simulink model "CurrentHysteresis_Control"  (R2023b)
settings: Solver=ode23  StartTime=0.0  StopTime=2  MaxStep=1e-5  RelTol=1e-3
model workspace: external: MATLAB File D:\Simulink\Study\PMSM建模第三章\CurrentHysteresis_Control_Params.m (data not in the file)
values from neighbouring files (symbols this model uses):
  B = 0.008    [CurrentHysteresis_Control_Params.m]    (also in Foc_Params.m; VF_Params.m)
  J = 0.0008    [CurrentHysteresis_Control_Params.m]    (also in Foc_Params.m = 0.003; VF_Params.m = 0.003)
  Pn = 4    [CurrentHysteresis_Control_Params.m]    (also in Foc_Params.m; VF_Params.m)
  R = 2.875    [CurrentHysteresis_Control_Params.m]    (also in Foc_Params.m = 0.958; VF_Params.m = 0.958)
libraries: spsControlledVoltageSourceLib x4, spsPermanentMagnetSynchronousMachineLib x2, slpidlib x1, sps_lib x1
settings Model: Creator=123  LastModifiedBy=123

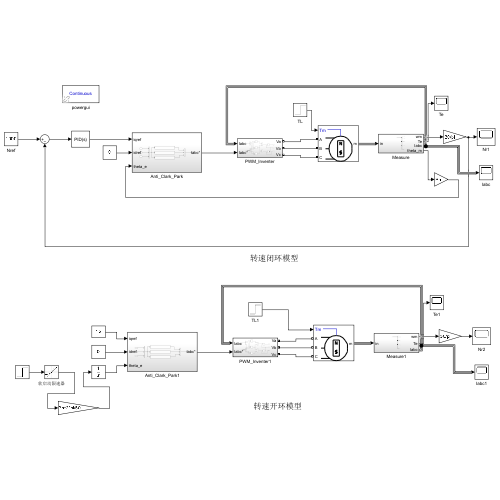
[thumbnail: Simulink's stored preview of the top-level diagram]
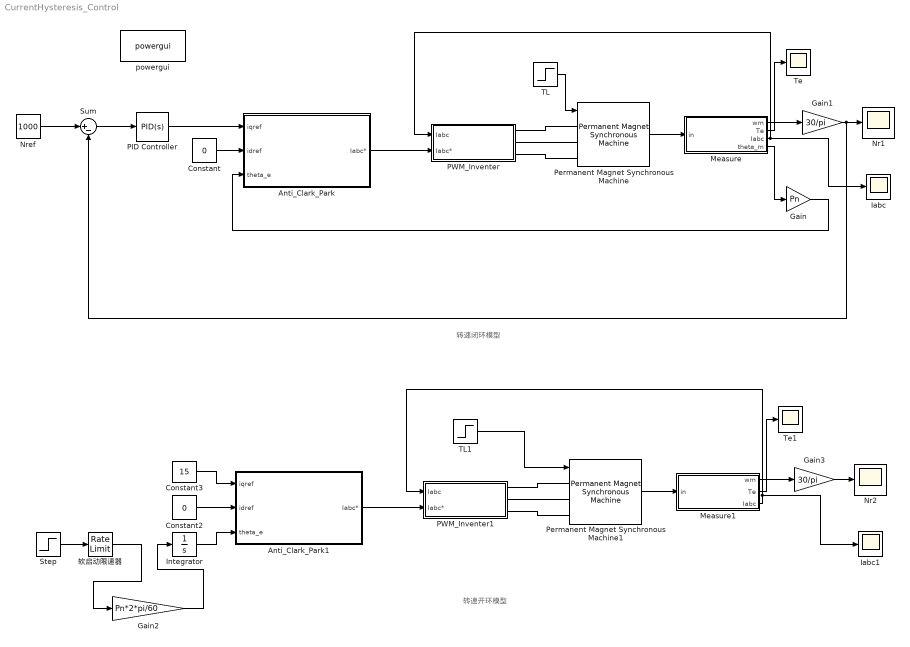
== system CurrentHysteresis_Control ==
  note: 转速开环模型
  note: 转速闭环模型
  Anti_Clark_Park : Subsystem
  Anti_Clark_Park1 : Subsystem
  Constant : Constant  Value=0
  Constant2 : Constant  Value=0
  Constant3 : Constant  Value=15
  Gain : Gain  Gain=Pn
  Gain1 : Gain  Gain=30/pi
  Gain2 : Gain  Gain=Pn*2*pi/60
  Gain3 : Gain  Gain=30/pi
  Iabc : Scope
  Iabc1 : Scope
  Integrator : Integrator
  Measure : Subsystem
  Measure1 : Subsystem
  Nr1 : Scope
  Nr2 : Scope
  Nref : Constant  Value=1000
  PID Controller : slpidlib/PID Controller  Controller=PID  Form=Parallel  TimeDomain=Continuous-time  UseExternalTs=off  SampleTime=-1  IntegratorMethod=Forward Euler  FilterMethod=Forward Euler  ControllerParametersSource=internal  P=0.06  I=10  UseKiTs=off  D=0  N=100  UseFilter=on  TunerSelectOption=Transfer Function Based (PID Tuner App)  InitialConditionSource=internal  InitialConditionForIntegrator=0  InitialConditionForFilter=0  DifferentiatorICPrevScaledInput=0  ExternalReset=none  TrackingMode=off  Kt=1  LimitOutput=off  SatLimitsSource=internal  UpperSaturationLimit=inf  LowerSaturationLimit=-inf  LinearizeAsGain=on  AntiWindupMode=none  Kb=1  LimitIntegrator=off  UpperIntegratorSaturationLimit=inf  LowerIntegratorSaturationLimit=-inf  POutMin=[]  POutMax=[]  IOutMin=[]  IOutMax=[]  DOutMin=[]  DOutMax=[]  NOutMin=[]  NOutMax=[]  SumOutMin=[]  SumOutMax=[]  SaturationOutMin=[]  SaturationOutMax=[]  PParamMin=[]  PParamMax=[]  IParamMin=[]  IParamMax=[]  DParamMin=[]  DParamMax=[]  NParamMin=[]  NParamMax=[]  KbParamMin=[]  KbParamMax=[]  KtParamMin=[]  KtParamMax=[]  KbOutMin=[]  KbOutMax=[]  KtOutMin=[]  KtOutMax=[]  IntegratorOutMin=[]  IntegratorOutMax=[]  FilterOutMin=[]  FilterOutMax=[]  SumI1OutMin=[]  SumI1OutMax=[]  SumI2OutMin=[]  SumI2OutMax=[]  SumI3OutMin=[]  SumI3OutMax=[]  SumI4OutMin=[]  SumI4OutMax=[]  SumDOutMin=[]  SumDOutMax=[]  DifferentiatorOutMin=[]  DifferentiatorOutMax=[]  FilterDiffOutCoefMin=[]  FilterDiffOutCoefMax=[]  ReciprocalOutMin=[]  ReciprocalOutMax=[]  SumDenOutMin=[]  SumDenOutMax=[]  SumNumOutMin=[]  SumNumOutMax=[]  DivideOutMin=[]  DivideOutMax=[]  UdiffTsProdOutMin=[]  UdiffTsProdOutMax=[]  NTsProdOutMin=[]  NTsProdOutMax=[]  UintegralTsProdOutMin=[]  UintegralTsProdOutMax=[]  UngainTsProdOutMin=[]  UngainTsProdOutMax=[]  ClampingZeroOutDataTypeStr=Inherit: Inherit via back propagation  ClampingZeroOutMin=[]  ClampingZeroOutMax=[]  FilterDenConstantOutDataTypeStr=Inherit: Inherit via back propagation  FilterDenConstantOutMin=[]  FilterDenConstantOutMax=[]  PCopyOutDataTypeStr=Inherit: Inherit via back propagation  PCopyOutMin=[]  PCopyOutMax=[]  NCopyOutDataTypeStr=Inherit: Inherit via back propagation  NCopyOutMin=[]  NCopyOutMax=[]  IntegratorContinuousStateAttributes=''  IntegratorStateMustResolveToSignalObject=off  IntegratorRTWStateStorageClass=Auto  FilterContinuousStateAttributes=''  FilterStateMustResolveToSignalObject=off  FilterRTWStateStorageClass=Auto  ParallelPVariant=InternalParameters  IdealPVariant=Disabled  IVariant=InternalParameters  DVariant=InternalParameters  IntegratorVariant=Continuous  SatVariant=Disabled  AWVariant=Passthrough  PCopyVariant=Disabled  TRVariant=Disabled  FdbkBlocksVariant=Forward  IdealPFdbkVariant=Disabled  SatFdbkVariant=Disabled  DerivativeFilterVariant=ContFilter  NVariant=InternalParameters  NCopyVariant=Disabled  FilterICVariant=InternalICsFilter  IntegratorICVariant=InternalICs  ExternalResetVariant=Disabled  TRSumVariant=Passthrough  SumFdbkVariant=Disabled  SumVariant=Sum_PID  TsampFilterVariant=InternalTs  TsampNgainVariant=Passthrough  TsampIntegralVariant=Disabled_SignalSpec  ExternalSaturationOutDataTypeStr=Inherit: Same as second input
  PWM_Inventer : Subsystem
  PWM_Inventer1 : Subsystem
  Permanent Magnet Synchronous Machine : spsPermanentMagnetSynchronousMachineLib/Permanent Magnet Synchronous Machine  NbPhases=3  FluxDistribution=Sinusoidal  RotorType=Round  MechanicalLoad=Torque Tm  PresetModel=No  ShowDetailedParameters=on  MeasurementBus=off  Resistance=R  Inductance=8.5e-3  dqInductances=[8.5e-3,8.5e-3]  La=Ld  MachineConstant=Flux linkage established by magnets (V.s)  Flux=flux  VoltageCst=126.966  TorqueCst=1.05  Flat=120  Mechanical=[J B Pn 0]  PolePairs=4  InitialConditions=[0,0, 0,0]  InitialConditions5ph=[0 0 0 0 0 0]  RefAngle=Aligned with phase A axis (original Park)  IterativeDiscreteModel=Trapezoidal non iterative  TsBlock=-1  TsPowergui=0
  Permanent Magnet Synchronous Machine1 : spsPermanentMagnetSynchronousMachineLib/Permanent Magnet Synchronous Machine  NbPhases=3  FluxDistribution=Sinusoidal  RotorType=Round  MechanicalLoad=Torque Tm  PresetModel=No  ShowDetailedParameters=on  MeasurementBus=off  Resistance=R  Inductance=8.5e-3  dqInductances=[8.5e-3,8.5e-3]  La=Ld  MachineConstant=Flux linkage established by magnets (V.s)  Flux=flux  VoltageCst=126.966  TorqueCst=1.05  Flat=120  Mechanical=[J B Pn 0]  PolePairs=4  InitialConditions=[0,0, 0,0]  InitialConditions5ph=[0 0 0 0 0 0]  RefAngle=Aligned with phase A axis (original Park)  IterativeDiscreteModel=Trapezoidal non iterative  TsBlock=-1  TsPowergui=0
  Step : Step  Time=0.1  After=1000  SampleTime=0
  Sum : Sum  Inputs=|+-
  TL : Step  Time=0.05  After=10  SampleTime=0
  TL1 : Step  After=10  SampleTime=0
  Te : Scope
  Te1 : Scope
  powergui : sps_lib/powergui  Priority=1  SimulationMode=Continuous  SampleTime=50e-6  frequency=60  Iterations=50  frequencyindice=0  Pbase=100e6  ErrMax=1e-4  UnitsV=kV  UnitsW=MW  buscounter=0  FunctionMessages=off  echomessages=off  EnableUseOfTLC=off  CurrentSourceSwitches=off  DisableSnubberDevices=off  DisableRonSwitches=off  DisableVfSwitches=off  DisplayEquations=off  AutomaticDiscreteSolvers=off  SolverType=Tustin/Backward Euler (TBE)  Interpol=off  ExternalGateDelay=off  methode=off  Ts=100  x0status=blocks  SPID=on  SwTol=0  HookPort=off  NonlinearTolerance=1e-4  nMaxIteration=100  ContinueOnMaxIteration=off  RestoreLinks=warning  ResistiveCurrentMeasurement=off  Frange=[0:2:500]  Ylog=off  Xlog=on  ShowGrid=off  save=off  variable=ZData  structure=0  ZoomFFT=off  StartTime=0.0  cycles=1  DisplayStyle=1  fundamental=60  FreqAxis=off  MaxFrequency=1000  frequencyindicesteady=1  RmsSteady=1  display=off
  软启动限速器 : RateLimiter  RisingSlewLimit=4000  FallingSlewLimit=-4000  SampleTimeMode=inherited
  wires:
  Nref/1 -> Sum/1
  Constant/1 -> Anti_Clark_Park/2(idref)
  Sum/1 -> PID Controller/1
  PID Controller/1 -> Anti_Clark_Park/1(iqref)
  Anti_Clark_Park/1(Iabc*) -> PWM_Inventer/2(Iabc*)
  Permanent Magnet Synchronous Machine/1 -> Measure/1(in)
  Gain1/1 -> Sum/2, Nr1/1
  Measure/1(wm) -> Gain1/1
  Measure/2(Te) -> Te/1
  Measure/4(theta_m) -> Gain/1
  Gain/1 -> Anti_Clark_Park/3(theta_e)
  Measure/3(Iabc) -> PWM_Inventer/1(Iabc), Iabc/1
  TL/1 -> Permanent Magnet Synchronous Machine/1
  Measure1/1(wm) -> Gain3/1
  Measure1/2(Te) -> Te1/1
  Gain3/1 -> Nr2/1
  Permanent Magnet Synchronous Machine1/1 -> Measure1/1(in)
  Measure1/3(Iabc) -> PWM_Inventer1/1(Iabc), Iabc1/1
  Anti_Clark_Park1/1(Iabc*) -> PWM_Inventer1/2(Iabc*)
  Step/1 -> 软启动限速器/1
  Integrator/1 -> Anti_Clark_Park1/3(theta_e)
  Constant2/1 -> Anti_Clark_Park1/2(idref)
  Constant3/1 -> Anti_Clark_Park1/1(iqref)
  软启动限速器/1 -> Gain2/1
  Gain2/1 -> Integrator/1
  TL1/1 -> Permanent Magnet Synchronous Machine1/1
  connections:
  PWM_Inventer/RConn1 -- Permanent Magnet Synchronous Machine/LConn1
  PWM_Inventer/RConn2 -- Permanent Magnet Synchronous Machine/LConn2
  PWM_Inventer/RConn3 -- Permanent Magnet Synchronous Machine/LConn3
  PWM_Inventer1/RConn3 -- Permanent Magnet Synchronous Machine1/LConn3
  PWM_Inventer1/RConn2 -- Permanent Magnet Synchronous Machine1/LConn2
  PWM_Inventer1/RConn1 -- Permanent Magnet Synchronous Machine1/LConn1

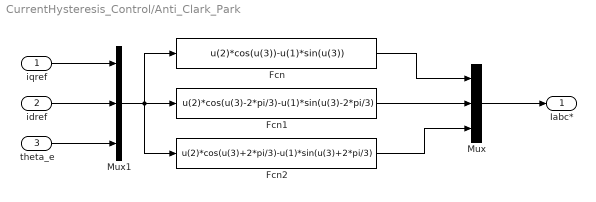
== system CurrentHysteresis_Control/Anti_Clark_Park ==
  iqref : Inport
  idref : Inport  Port=2
  theta_e : Inport  Port=3
  Fcn : Fcn  Expr=u(2)*cos(u(3))-u(1)*sin(u(3))
  Fcn1 : Fcn  Expr=u(2)*cos(u(3)-2*pi/3)-u(1)*sin(u(3)-2*pi/3)
  Fcn2 : Fcn  Expr=u(2)*cos(u(3)+2*pi/3)-u(1)*sin(u(3)+2*pi/3)
  Mux : Mux  Inputs=3
  Mux1 : Mux  Inputs=3
  Iabc* : Outport
  wires:
  Mux/1 -> Iabc*/1
  Fcn/1 -> Mux/1
  Fcn1/1 -> Mux/2
  Fcn2/1 -> Mux/3
  iqref/1 -> Mux1/1
  idref/1 -> Mux1/2
  theta_e/1 -> Mux1/3
  Mux1/1 -> Fcn1/1, Fcn/1, Fcn2/1

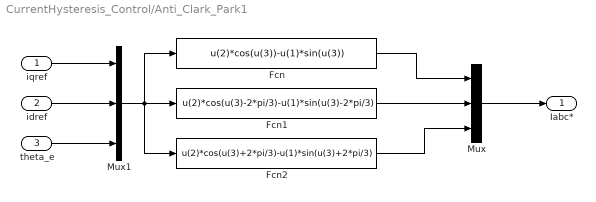
== system CurrentHysteresis_Control/Anti_Clark_Park1 ==
  iqref : Inport
  idref : Inport  Port=2
  theta_e : Inport  Port=3
  Fcn : Fcn  Expr=u(2)*cos(u(3))-u(1)*sin(u(3))
  Fcn1 : Fcn  Expr=u(2)*cos(u(3)-2*pi/3)-u(1)*sin(u(3)-2*pi/3)
  Fcn2 : Fcn  Expr=u(2)*cos(u(3)+2*pi/3)-u(1)*sin(u(3)+2*pi/3)
  Mux : Mux  Inputs=3
  Mux1 : Mux  Inputs=3
  Iabc* : Outport
  wires:
  Mux/1 -> Iabc*/1
  Fcn/1 -> Mux/1
  Fcn1/1 -> Mux/2
  Fcn2/1 -> Mux/3
  iqref/1 -> Mux1/1
  idref/1 -> Mux1/2
  theta_e/1 -> Mux1/3
  Mux1/1 -> Fcn1/1, Fcn/1, Fcn2/1

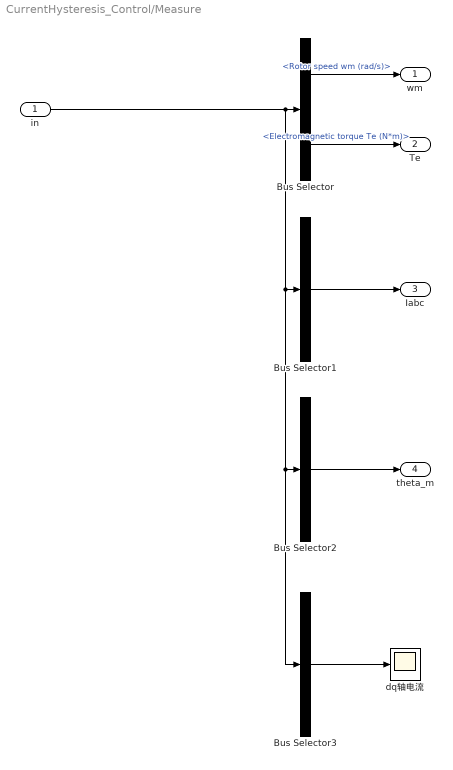
== system CurrentHysteresis_Control/Measure ==
  in : Inport
  Bus Selector : BusSelector  OutputSignals=Rotor speed wm (rad/s),Electromagnetic torque Te (N*m)
  Bus Selector1 : BusSelector  OutputSignals=Stator current is_a (A),Stator current is_b (A),Stator current is_c (A)  OutputAsBus=on
  Bus Selector2 : BusSelector  OutputSignals=Rotor angle thetam (rad)  OutputAsBus=on
  Bus Selector3 : BusSelector  OutputSignals=Stator current is_d (A),Stator current is_q (A)  OutputAsBus=on
  dq轴电流 : Scope
  wm : Outport
  Te : Outport  Port=2
  Iabc : Outport  Port=3
  theta_m : Outport  Port=4
  wires:
  in/1 -> Bus Selector3/1, Bus Selector2/1, Bus Selector1/1, Bus Selector/1
  Bus Selector/1 -> wm/1  "<Rotor speed wm (rad/s)>"
  Bus Selector/2 -> Te/1  "<Electromagnetic torque Te (N*m)>"
  Bus Selector1/1 -> Iabc/1
  Bus Selector2/1 -> theta_m/1
  Bus Selector3/1 -> dq轴电流/1

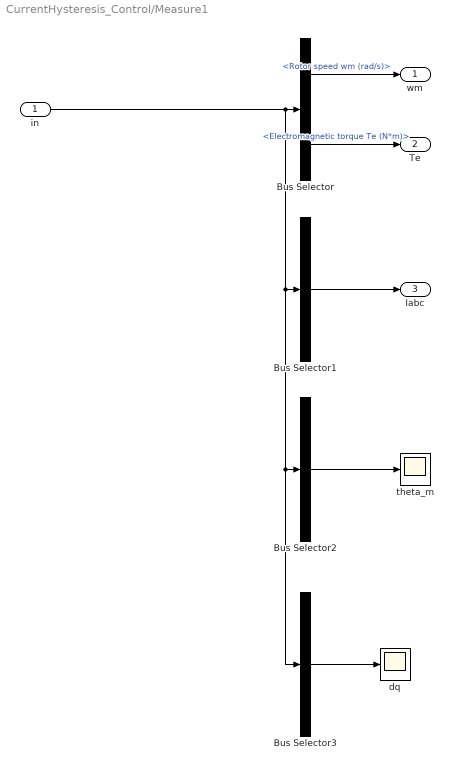
== system CurrentHysteresis_Control/Measure1 ==
  in : Inport
  Bus Selector : BusSelector  OutputSignals=Rotor speed wm (rad/s),Electromagnetic torque Te (N*m)
  Bus Selector1 : BusSelector  OutputSignals=Stator current is_a (A),Stator current is_b (A),Stator current is_c (A)  OutputAsBus=on
  Bus Selector2 : BusSelector  OutputSignals=Rotor angle thetam (rad)  OutputAsBus=on
  Bus Selector3 : BusSelector  OutputSignals=Stator current is_d (A),Stator current is_q (A)  OutputAsBus=on
  dq : Scope
  theta_m : Scope
  wm : Outport
  Te : Outport  Port=2
  Iabc : Outport  Port=3
  wires:
  in/1 -> Bus Selector3/1, Bus Selector2/1, Bus Selector1/1, Bus Selector/1
  Bus Selector/1 -> wm/1  "<Rotor speed wm (rad/s)>"
  Bus Selector/2 -> Te/1  "<Electromagnetic torque Te (N*m)>"
  Bus Selector1/1 -> Iabc/1
  Bus Selector2/1 -> theta_m/1
  Bus Selector3/1 -> dq/1

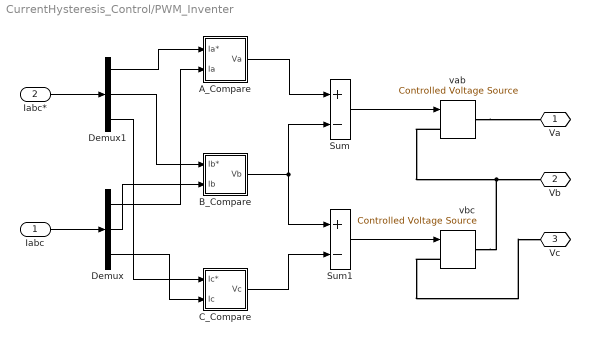
== system CurrentHysteresis_Control/PWM_Inventer ==
  Iabc : Inport
  Iabc* : Inport  Port=2
  A_Compare : Subsystem
  B_Compare : Subsystem
  C_Compare : Subsystem
  Demux : Demux  Outputs=3
  Demux1 : Demux  Outputs=3
  Sum : Sum  Inputs=+-
  Sum1 : Sum  Inputs=+-
  vab : spsControlledVoltageSourceLib/Controlled Voltage Source  Initialize=on  Source_Type=AC  Amplitude=0  Phase=0  Frequency=0  Measurements=None
  vbc : spsControlledVoltageSourceLib/Controlled Voltage Source  Initialize=on  Source_Type=AC  Amplitude=0  Phase=0  Frequency=0  Measurements=None
  Va : PMIOPort  Side=Right
  Vb : PMIOPort  Port=2  Side=Right
  Vc : PMIOPort  Port=3  Side=Right
  wires:
  Iabc/1 -> Demux/1
  Iabc*/1 -> Demux1/1
  Demux1/1 -> A_Compare/1(Ia*)
  Demux1/2 -> B_Compare/1(Ib*)
  Demux1/3 -> C_Compare/1(Ic*)
  Demux/3 -> C_Compare/2(Ic)
  Demux/2 -> B_Compare/2(Ib)
  Demux/1 -> A_Compare/2(Ia)
  A_Compare/1(Va) -> Sum/1
  B_Compare/1(Vb) -> Sum1/1, Sum/2
  C_Compare/1(Vc) -> Sum1/2
  Sum/1 -> vab/1
  Sum1/1 -> vbc/1
  connections:
  vab/RConn1 -- Va/RConn1
  vab/LConn1 -- vbc/RConn1 -- Vb/RConn1
  vbc/LConn1 -- Vc/RConn1

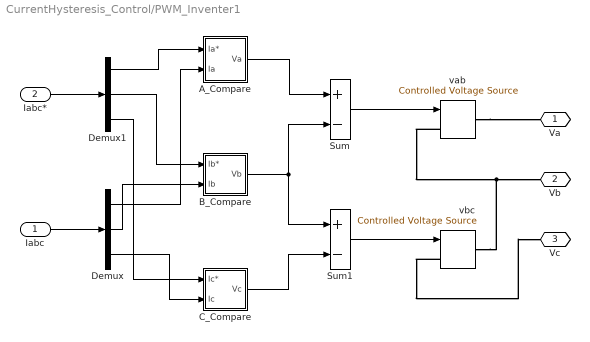
== system CurrentHysteresis_Control/PWM_Inventer1 ==
  Iabc : Inport
  Iabc* : Inport  Port=2
  A_Compare : Subsystem
  B_Compare : Subsystem
  C_Compare : Subsystem
  Demux : Demux  Outputs=3
  Demux1 : Demux  Outputs=3
  Sum : Sum  Inputs=+-
  Sum1 : Sum  Inputs=+-
  vab : spsControlledVoltageSourceLib/Controlled Voltage Source  Initialize=on  Source_Type=AC  Amplitude=0  Phase=0  Frequency=0  Measurements=None
  vbc : spsControlledVoltageSourceLib/Controlled Voltage Source  Initialize=on  Source_Type=AC  Amplitude=0  Phase=0  Frequency=0  Measurements=None
  Va : PMIOPort  Side=Right
  Vb : PMIOPort  Port=2  Side=Right
  Vc : PMIOPort  Port=3  Side=Right
  wires:
  Iabc/1 -> Demux/1
  Iabc*/1 -> Demux1/1
  Demux1/1 -> A_Compare/1(Ia*)
  Demux1/2 -> B_Compare/1(Ib*)
  Demux1/3 -> C_Compare/1(Ic*)
  Demux/3 -> C_Compare/2(Ic)
  Demux/2 -> B_Compare/2(Ib)
  Demux/1 -> A_Compare/2(Ia)
  A_Compare/1(Va) -> Sum/1
  B_Compare/1(Vb) -> Sum1/1, Sum/2
  C_Compare/1(Vc) -> Sum1/2
  Sum/1 -> vab/1
  Sum1/1 -> vbc/1
  connections:
  vab/RConn1 -- Va/RConn1
  vab/LConn1 -- vbc/RConn1 -- Vb/RConn1
  vbc/LConn1 -- Vc/RConn1

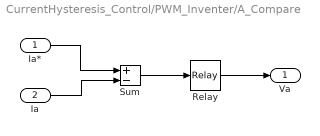
== system CurrentHysteresis_Control/PWM_Inventer/A_Compare ==
  Ia* : Inport
  Ia : Inport  Port=2
  Relay : Relay  OnSwitchValue=0.05  OffSwitchValue=-0.05  OnOutputValue=150  OffOutputValue=-150
  Sum : Sum  Inputs=+-
  Va : Outport
  wires:
  Sum/1 -> Relay/1
  Ia*/1 -> Sum/1
  Relay/1 -> Va/1
  Ia/1 -> Sum/2

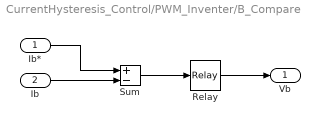
== system CurrentHysteresis_Control/PWM_Inventer/B_Compare ==
  Ib* : Inport
  Ib : Inport  Port=2
  Relay : Relay  OnSwitchValue=0.05  OffSwitchValue=-0.05  OnOutputValue=150  OffOutputValue=-150
  Sum : Sum  Inputs=+-
  Vb : Outport
  wires:
  Sum/1 -> Relay/1
  Ib*/1 -> Sum/1
  Relay/1 -> Vb/1
  Ib/1 -> Sum/2

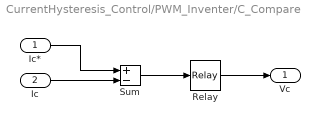
== system CurrentHysteresis_Control/PWM_Inventer/C_Compare ==
  Ic* : Inport
  Ic : Inport  Port=2
  Relay : Relay  OnSwitchValue=0.05  OffSwitchValue=-0.05  OnOutputValue=150  OffOutputValue=-150
  Sum : Sum  Inputs=+-
  Vc : Outport
  wires:
  Sum/1 -> Relay/1
  Ic*/1 -> Sum/1
  Relay/1 -> Vc/1
  Ic/1 -> Sum/2

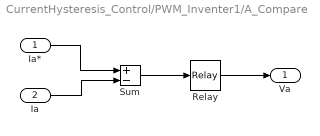
== system CurrentHysteresis_Control/PWM_Inventer1/A_Compare ==
  Ia* : Inport
  Ia : Inport  Port=2
  Relay : Relay  OnSwitchValue=0.05  OffSwitchValue=-0.05  OnOutputValue=150  OffOutputValue=-150
  Sum : Sum  Inputs=+-
  Va : Outport
  wires:
  Sum/1 -> Relay/1
  Ia*/1 -> Sum/1
  Relay/1 -> Va/1
  Ia/1 -> Sum/2

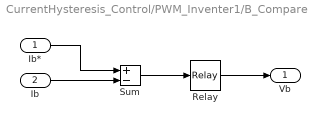
== system CurrentHysteresis_Control/PWM_Inventer1/B_Compare ==
  Ib* : Inport
  Ib : Inport  Port=2
  Relay : Relay  OnSwitchValue=0.05  OffSwitchValue=-0.05  OnOutputValue=150  OffOutputValue=-150
  Sum : Sum  Inputs=+-
  Vb : Outport
  wires:
  Sum/1 -> Relay/1
  Ib*/1 -> Sum/1
  Relay/1 -> Vb/1
  Ib/1 -> Sum/2

== system CurrentHysteresis_Control/PWM_Inventer1/C_Compare ==
  Ic* : Inport
  Ic : Inport  Port=2
  Relay : Relay  OnSwitchValue=0.05  OffSwitchValue=-0.05  OnOutputValue=150  OffOutputValue=-150
  Sum : Sum  Inputs=+-
  Vc : Outport
  wires:
  Sum/1 -> Relay/1
  Ic*/1 -> Sum/1
  Relay/1 -> Vc/1
  Ic/1 -> Sum/2
